simulink model "RobustFormationControl_FractionalModel_under_Dis"  (R2023a)
settings: Solver=ode3  StartTime=0.0  StopTime=30  FixedStep=0.0001  RelTol=1e-3
InitFcn:
  | % close all;
  | % clear all;
  | % clc;
  | % System & Qaudrotor Parameters
  | %==============================
  | m = 0.486;                                         % Quadrotor Mass ( kg )
  | 
  | L = 0.25;                                         % Length of the arm ( m )
  | % L = 0.25;                                         % Length of the arm ( m )
  | 
  | Ixx = 4.856e-03; Iyy = 4.856e-03; Izz = 8.801e-03; % The moments of inertia around x,y and z axes respectively ( kg.m^2 )
  | % Ixx = 3.8278e-03; Iyy = 3.8278e-03; Izz = 7.6566e-03; % The moments of inertia around x,y and z axes respectively ( kg.m^2 )
  | 
  | Jr = 2.8385e-5;                                            % The inertia moment of rotor ( kg.m^2 )
  | % Jr = 0;
  | 
  | % Kx=5.5670e-4;
  | % Ky=5.5670e-4;
  | % Kz=6.3540e-4;
  | % kx=0.032;
  | % ky=0.032;
  | % kz=0.048;
  | Kfx = 5.5670e-4; Kfy = 5.5670e-4; Kfz = 6.3540e-4;% The Rotational drag cofficients ( N/rad/s )
  | 
  | % Ktx = 0.032; Kty = 0.032; Ktz = 0.048;               % The linear drag coefficients in x, y, z respectively ( N/m/s )
  | Ktx = 5.5670e-4; Kty =5.5670e-4; Ktz = 6.3540e-4;               % The linear drag coefficients in x, y, z respectively ( N/m/s )
  | 
  | b = 2.923e-05;                                      % The lift coefficient
  | % b = 2.9842e-05;                                      % The lift coefficient
  | 
  | d = 1.12e-06;                                       % The drag coefficient
  | % d = 3.2320e-07;                                       % The drag coefficient
  | 
  | g = 9.81;                                          % The acceleration due to gravity ( m/s^2 )
  | 
  | %-------- The Coefficients of Non-linear Equations of Quadrotor ( Page 11) -------
  | %--------------------------------------------------------------------------------
  | % Rotational Equations
  | %=====================
  | % Coefficients in ( eq1 ) >>..
  | a1 = (Iyy - Izz)/Ixx;
  | b1 = - Jr/Ixx;
  | c1 = - Kfx/Ixx;
  | d1 = L/Ixx;
  | 
  | % Coefficients in ( eq2 ) >>..
  | a2 = (Izz - Ixx)/Iyy;
  | b2 = Jr/Iyy;
  | c2 = - Kfy/Iyy;
  | d2 = L/Iyy;
  | 
  | % Coefficients in ( eq3 ) >>..
  | a3 = (Ixx - Iyy)/Izz;
  | b3 = - Kfz/Izz;
  | c3 = 1/Izz;
  | % c3 = d/Izz;
  | 
  | % Translational Equations
  | %========================
  | % Coefficients in ( eq4 ) >>..
  | ... (+151 lines)
libraries: fod x135, eeStairGenerator x5
(part 9 of 10)

== system RobustFormationControl_FractionalModel_under_Dis/Fractional Leader with four followers/Follower 4 System/Follower 2 Quadrotor Model/Control Module1/Subsystem5/Subsystem2 ==
  x5 : Inport
  xd5 : Inport  Port=2
  x6 : Inport  Port=3
  xd6 : Inport  Port=4
  S6 : Inport  Port=5
  Abs : Abs  SaturateOnIntegerOverflow=off
  Divide{,1..4} (5 alike) : Product  Inputs=**  RndMeth=Zero  SaturateOnIntegerOverflow=on
  Gain : Gain  Gain=q0
  Gain1 : Gain  Gain=q1
  Gain2 : Gain  Gain=q2
  Integrator : Integrator
  Integrator1 : Integrator
  Integrator2 : Integrator
  Sum1 : Sum  Inputs=+-
  Sum2 : Sum  Inputs=----
  Sum3 : Sum  Inputs=+-
  Tanh : Trigonometry  Operator=tanh
  w : Constant  Value=w
  D3 : Outport  VectorParamsAs1DForOutWhenUnconnected=off
  wires:
  xd6/1 -> Sum1/2
  xd5/1 -> Sum3/2
  x5/1 -> Sum3/1
  x6/1 -> Sum1/1
  S6/1 -> [S6], Abs/1
  Sum1/1 -> [e2]
  Sum3/1 -> [e1]
  Gain/1 -> Integrator/1
  Integrator/1 -> Sum2/1  "B0"
  [e1] -> Divide/2
  Gain1/1 -> Integrator1/1
  Divide/1 -> Gain1/1
  Divide1/1 -> Gain2/1
  Gain2/1 -> Integrator2/1
  [e2] -> Divide1/2
  Abs/1 -> Divide1/1, Divide/1, Gain/1
  Integrator1/1 -> Divide3/2  "B1"
  w/1 -> Sum2/4
  Tanh/1 -> Divide2/2
  [S6] -> Tanh/1
  Divide2/1 -> D3/1
  [e1] -> Divide3/1
  [e2] -> Divide4/1
  Integrator2/1 -> Divide4/2  "B2"
  Divide3/1 -> Sum2/2
  Divide4/1 -> Sum2/3
  Sum2/1 -> Divide2/1

== system RobustFormationControl_FractionalModel_under_Dis/Fractional Leader with four followers/Follower 4 System/Follower 2 Quadrotor Model/Control Module1/Subsystem6/Subsystem3 ==
  xL : Inport
  x7 : Inport  Port=2
  x8 : Inport  Port=3
  dX : Inport  Port=4
  S8 : Inport  Port=5
  Constant : Constant  Value=p/q
  Constant1 : Constant  Value=gx-1
  Derivative : Derivative
  Derivative1 : Derivative
  Divide : Product  Inputs=**  RndMeth=Zero  SaturateOnIntegerOverflow=on
  Fractional derivative : fod/Fractional derivative  gam=alpha1(1)  ww=[0.001; 1000]  n=5  nFod=off
      settings: SourceProductName=FOMCON Toolbox
  Fractional integrator1 : fod/Fractional integrator  gam=alpha2(1)  ww=[0.001; 1000]  n=5  nFod=off
      settings: SourceProductName=FOMCON Toolbox
  Gain : Gain  Gain=cx1
  Gain1 : Gain  Gain=cx2
  Gain2 : Gain  Gain=gx
  Gain3 : Gain  Gain=Sigma1X
  Gain4 : Gain  Gain=Sigma2X
  Power : Math  Operator=pow
  Power1 : Math  Operator=pow
  Sum : Sum
  Sum1 : Sum  Inputs=+--
  Sum2 : Sum  Inputs=+++
  Sum3 : Sum  Inputs=+--
  Tanh : Trigonometry  Operator=tanh
  D2 : Outport  VectorParamsAs1DForOutWhenUnconnected=off
  wires:
  Sum3/1 -> Power1/1, Power/1
  Constant/1 -> Power/2
  Power/1 -> Gain/1
  Gain/1 -> Fractional derivative/1
  Constant1/1 -> Power1/2
  Power1/1 -> Divide/2
  Divide/1 -> Gain1/1
  Gain1/1 -> Gain2/1
  Sum1/1 -> Divide/1
  Gain2/1 -> Fractional integrator1/1
  S8/1 -> Tanh/1, Gain4/1
  Tanh/1 -> Gain3/1
  Gain3/1 -> Sum/1
  Gain4/1 -> Sum/2
  Sum/1 -> Sum2/3
  Fractional derivative/1 -> Sum2/1
  Fractional integrator1/1 -> Sum2/2
  Sum2/1 -> D2/1
  xL/1 -> Sum3/1, Derivative/1
  Derivative/1 -> Sum1/1
  x8/1 -> Sum1/2
  dX/1 -> Sum3/3, Derivative1/1
  Derivative1/1 -> Sum1/3
  x7/1 -> Sum3/2

== system RobustFormationControl_FractionalModel_under_Dis/Fractional Leader with four followers/Follower 4 System/Follower 2 Quadrotor Model/Control Module1/Subsystem6/Subsystem4 ==
  x8 : Inport
  xL : Inport  Port=2
  dX : Inport  Port=3
  Derivative{,1..3} (4 alike) : Derivative
  Divide2 : Product  Inputs=**  RndMeth=Zero  SaturateOnIntegerOverflow=on
  Gain1 : Gain  Commented=on  Gain=a6
  Sum : Sum  Inputs=-+-
  D1 : Outport
  wires:
  Sum/1 -> D1/1
  x8/1 -> Divide2/2
  Divide2/1 -> Sum/1
  [a4D] -> Divide2/1
  Derivative/1 -> Derivative1/1
  xL/1 -> Derivative/1
  Derivative3/1 -> Sum/3
  Derivative2/1 -> Derivative3/1
  dX/1 -> Derivative2/1
  Derivative1/1 -> Sum/2

== system RobustFormationControl_FractionalModel_under_Dis/Fractional Leader with four followers/Follower 4 System/Follower 2 Quadrotor Model/Control Module1/Subsystem6/Subsystem5 ==
  xL : Inport
  x7 : Inport  Port=2
  x8 : Inport  Port=3
  dX : Inport  Port=4
  S8 : Inport  Port=5
  Abs : Abs  SaturateOnIntegerOverflow=off
  Derivative : Derivative
  Derivative1 : Derivative
  Divide{,1..4} (5 alike) : Product  Inputs=**  RndMeth=Zero  SaturateOnIntegerOverflow=on
  Gain : Gain  Gain=q0
  Gain1 : Gain  Gain=q1
  Gain2 : Gain  Gain=q2
  Integrator : Integrator
  Integrator1 : Integrator
  Integrator2 : Integrator
  Sum2 : Sum  Inputs=++++
  Sum4 : Sum  Inputs=+--
  Sum5 : Sum  Inputs=+--
  Tanh : Trigonometry  Operator=tanh
  w : Constant  Value=w
  D3 : Outport  VectorParamsAs1DForOutWhenUnconnected=off
  wires:
  S8/1 -> [S8], Abs/1
  Gain/1 -> Integrator/1
  Integrator/1 -> Sum2/1  "B0"
  [e1] -> Divide/2
  Gain1/1 -> Integrator1/1
  Divide/1 -> Gain1/1
  Divide1/1 -> Gain2/1
  Gain2/1 -> Integrator2/1
  [e2] -> Divide1/2
  Abs/1 -> Divide1/1, Divide/1, Gain/1
  Integrator1/1 -> Divide3/2  "B1"
  w/1 -> Sum2/4
  Tanh/1 -> Divide2/2
  [S8] -> Tanh/1
  Divide2/1 -> D3/1
  [e1] -> Divide3/1
  [e2] -> Divide4/1
  Integrator2/1 -> Divide4/2  "B2"
  Divide3/1 -> Sum2/2
  Divide4/1 -> Sum2/3
  Sum2/1 -> Divide2/1
  Derivative1/1 -> Sum4/3
  Derivative/1 -> Sum4/1
  Sum4/1 -> [e2]
  Sum5/1 -> [e1]
  xL/1 -> Sum5/1, Derivative/1
  x8/1 -> Sum4/2
  dX/1 -> Sum5/3, Derivative1/1
  x7/1 -> Sum5/2

== system RobustFormationControl_FractionalModel_under_Dis/Fractional Leader with four followers/Follower 4 System/Follower 2 Quadrotor Model/Control Module1/Subsystem8/Subsystem ==
  x3 : Inport
  xd3 : Inport  Port=2
  x4 : Inport  Port=3
  xd4 : Inport  Port=4
  S4 : Inport  Port=5
  Constant : Constant  Value=p/q
  Constant1 : Constant  Value=gammaP(2)-1
  Divide : Product  Inputs=**  RndMeth=Zero  SaturateOnIntegerOverflow=on
  Fractional derivative : fod/Fractional derivative  gam=alpha1(2)  ww=[0.001; 1000]  n=5  nFod=off
      settings: SourceProductName=FOMCON Toolbox
  Fractional integrator1 : fod/Fractional integrator  gam=alpha2(2)  ww=[0.001; 1000]  n=5  nFod=off
      settings: SourceProductName=FOMCON Toolbox
  Gain : Gain  Gain=cTheta1
  Gain1 : Gain  Gain=cTheta2
  Gain2 : Gain  Gain=gammaP(2)
  Gain3 : Gain  Gain=Sigma1Theta
  Gain4 : Gain  Gain=Sigma2Theta
  Power : Math  Operator=pow
  Power1 : Math  Operator=pow
  Sum : Sum
  Sum1 : Sum  Inputs=+-
  Sum2 : Sum  Inputs=---
  Sum3 : Sum  Inputs=+-
  Tanh : Trigonometry  Operator=tanh
  D2 : Outport  VectorParamsAs1DForOutWhenUnconnected=off
  wires:
  xd4/1 -> Sum1/2
  xd3/1 -> Sum3/2
  x3/1 -> Sum3/1
  x4/1 -> Sum1/1
  Sum3/1 -> Power1/1, Power/1
  Constant/1 -> Power/2
  Power/1 -> Gain/1
  Gain/1 -> Fractional derivative/1
  Constant1/1 -> Power1/2
  Power1/1 -> Divide/2
  Divide/1 -> Gain1/1
  Gain1/1 -> Gain2/1
  Sum1/1 -> Divide/1
  Gain2/1 -> Fractional integrator1/1
  S4/1 -> Tanh/1, Gain4/1
  Tanh/1 -> Gain3/1
  Gain3/1 -> Sum/1
  Gain4/1 -> Sum/2
  Sum/1 -> Sum2/3
  Fractional derivative/1 -> Sum2/1
  Fractional integrator1/1 -> Sum2/2
  Sum2/1 -> D2/1

== system RobustFormationControl_FractionalModel_under_Dis/Fractional Leader with four followers/Follower 4 System/Follower 2 Quadrotor Model/Control Module1/Subsystem8/Subsystem1 ==
  x4 : Inport
  x6 : Inport  Port=2
  x2 : Inport  Port=3
  Omega : Inport  Port=4
  xd4 : Inport  Port=5
  Gain1 : Gain  Gain=a2
  Gain2 : Gain  Gain=c2
  Gain3 : Gain  Gain=b2
  Math Function1 : Math  Operator=square  SignedPower=on
  Product2 : Product
  Product4 : Product
  Sum3 : Sum  Inputs=---+
  D1 : Outport
  wires:
  x6/1 -> Product2/2
  Gain1/1 -> Sum3/1  "a1 x4 x6"
  Sum3/1 -> D1/1
  Math Function1/1 -> Gain2/1  "x2^2"
  x2/1 -> Product4/1, Product2/1
  x4/1 -> Math Function1/1
  xd4/1 -> Sum3/4
  Product4/1 -> Gain3/1
  Omega/1 -> Product4/2
  Product2/1 -> Gain1/1
  Gain3/1 -> Sum3/3
  Gain2/1 -> Sum3/2  "c1 x2^2"

== system RobustFormationControl_FractionalModel_under_Dis/Fractional Leader with four followers/Follower 4 System/Follower 2 Quadrotor Model/Control Module1/Subsystem8/Subsystem2 ==
  x3 : Inport
  xd3 : Inport  Port=2
  x4 : Inport  Port=3
  xd4 : Inport  Port=4
  S4 : Inport  Port=5
  Abs : Abs  SaturateOnIntegerOverflow=off
  Divide{,1..4} (5 alike) : Product  Inputs=**  RndMeth=Zero  SaturateOnIntegerOverflow=on
  Gain : Gain  Gain=q0
  Gain1 : Gain  Gain=q1
  Gain2 : Gain  Gain=q2
  Integrator : Integrator
  Integrator1 : Integrator
  Integrator2 : Integrator
  Sum1 : Sum  Inputs=+-
  Sum2 : Sum  Inputs=----
  Sum3 : Sum  Inputs=+-
  Tanh : Trigonometry  Operator=tanh
  w : Constant  Value=w
  D3 : Outport  VectorParamsAs1DForOutWhenUnconnected=off
  wires:
  xd4/1 -> Sum1/2
  xd3/1 -> Sum3/2
  x3/1 -> Sum3/1
  x4/1 -> Sum1/1
  S4/1 -> [S4], Abs/1
  Sum1/1 -> [e2]
  Sum3/1 -> [e1]
  Gain/1 -> Integrator/1
  Integrator/1 -> Sum2/1  "B0"
  [e1] -> Divide/2
  Gain1/1 -> Integrator1/1
  Divide/1 -> Gain1/1
  Divide1/1 -> Gain2/1
  Gain2/1 -> Integrator2/1
  [e2] -> Divide1/2
  Abs/1 -> Divide1/1, Divide/1, Gain/1
  Integrator1/1 -> Divide3/2  "B1"
  w/1 -> Sum2/4
  Tanh/1 -> Divide2/2
  [S4] -> Tanh/1
  Divide2/1 -> D3/1
  [e1] -> Divide3/1
  [e2] -> Divide4/1
  Integrator2/1 -> Divide4/2  "B2"
  Divide3/1 -> Sum2/2
  Divide4/1 -> Sum2/3
  Sum2/1 -> Divide2/1

== system RobustFormationControl_FractionalModel_under_Dis/Fractional Leader with four followers/Follower 4 System/Follower 2 Quadrotor Model/Quadrotor Dynamic System/Rotational System/Equation1 ==
  x4 : Inport
  x6 : Inport  Port=2
  U2 : Inport  Port=3
  Omega : Inport  Port=4
  Gain : Gain  Gain=a1
  Gain1 : Gain  Gain=c1
  Gain2 : Gain  Gain=b1
  Gain3 : Gain  Gain=d1
  Integrator : Integrator
  Integrator1 : Integrator
  Math Function : Math  Operator=square  SignedPower=on
  Product : Product
  Product1 : Product
  Sum : Sum  Inputs=|++++
  x1 = Phi : Outport  VectorParamsAs1DForOutWhenUnconnected=off
  x2 : Outport  Port=2  VectorParamsAs1DForOutWhenUnconnected=off
  wires:
  Math Function/1 -> Gain1/1  "x2^2"
  x4/1 -> Product1/1, Product/1
  Integrator/1 -> Math Function/1, x2/1, Integrator1/1
  U2/1 -> Gain3/1
  Gain2/1 -> Sum/3
  Gain3/1 -> Sum/4
  Gain/1 -> Sum/1  "a1 x4 x6"
  Product1/1 -> Gain2/1
  Gain1/1 -> Sum/2  "c1 x2^2"
  Integrator1/1 -> x1 = Phi/1
  Product/1 -> Gain/1
  x6/1 -> Product/2
  Sum/1 -> Integrator/1
  Omega/1 -> Product1/2

== system RobustFormationControl_FractionalModel_under_Dis/Fractional Leader with four followers/Follower 4 System/Follower 2 Quadrotor Model/Quadrotor Dynamic System/Rotational System/Equation2 ==
  x2 : Inport
  x6 : Inport  Port=2
  U3 : Inport  Port=3
  Omega : Inport  Port=4
  Gain : Gain  Gain=a2
  Gain1 : Gain  Gain=c2
  Gain2 : Gain  Gain=b2
  Gain3 : Gain  Gain=d2
  Integrator : Integrator
  Integrator1 : Integrator
  Math Function : Math  Operator=square  SignedPower=on
  Product : Product
  Product1 : Product
  Sum : Sum  Inputs=|++++
  x3 =Theta : Outport  VectorParamsAs1DForOutWhenUnconnected=off
  x4 : Outport  Port=2  VectorParamsAs1DForOutWhenUnconnected=off
  wires:
  Math Function/1 -> Gain1/1  "x4^2"
  x2/1 -> Product1/1, Product/1
  Integrator/1 -> Math Function/1, x4/1, Integrator1/1
  U3/1 -> Gain3/1
  Gain2/1 -> Sum/3
  Gain3/1 -> Sum/4
  Gain/1 -> Sum/1  "a2 x2 x6"
  Product1/1 -> Gain2/1
  Gain1/1 -> Sum/2  "c2 x2^2"
  Integrator1/1 -> x3 =Theta/1
  Product/1 -> Gain/1
  x6/1 -> Product/2
  Sum/1 -> Integrator/1
  Omega/1 -> Product1/2

== system RobustFormationControl_FractionalModel_under_Dis/Fractional Leader with four followers/Follower 4 System/Follower 2 Quadrotor Model/Quadrotor Dynamic System/Rotational System/Equation3 ==
  x2 : Inport
  x4 : Inport  Port=2
  U4 : Inport  Port=3
  Gain : Gain  Gain=a3
  Gain1 : Gain  Gain=b3
  Gain3 : Gain  Gain=c3
  Integrator : Integrator
  Integrator1 : Integrator
  Math Function : Math  Operator=square  SignedPower=on
  Product : Product
  Sum : Sum  Inputs=|+++
  x5 =Psi : Outport  VectorParamsAs1DForOutWhenUnconnected=off
  x6 : Outport  Port=2  VectorParamsAs1DForOutWhenUnconnected=off
  wires:
  Math Function/1 -> Gain1/1  "x6^2"
  x2/1 -> Product/1
  Integrator/1 -> Math Function/1, x6/1, Integrator1/1
  U4/1 -> Gain3/1
  Gain3/1 -> Sum/3
  Gain/1 -> Sum/1  "a3 x2 x4"
  Gain1/1 -> Sum/2  "b3 x6^2"
  Integrator1/1 -> x5 =Psi/1
  Product/1 -> Gain/1
  x4/1 -> Product/2
  Sum/1 -> Integrator/1

== system RobustFormationControl_FractionalModel_under_Dis/Fractional Leader with four followers/Follower 4 System/Follower 2 Quadrotor Model/Quadrotor Dynamic System/Translational System/Equation4 ==
  U1 : Inport
  Ux : Inport  Port=2
  Gain : Gain  Gain=1/m
  Gain1 : Gain  Gain=a4
  Integrator : Integrator
  Integrator1 : Integrator  InitialCondition=4
  Product : Product
  Sum : Sum  Inputs=|++
  x7 = x : Outport  VectorParamsAs1DForOutWhenUnconnected=off
  x8 = xdot : Outport  Port=2  VectorParamsAs1DForOutWhenUnconnected=off
  wires:
  Integrator/1 -> Gain1/1, x8 = xdot/1, Integrator1/1
  U1/1 -> Product/1
  Gain/1 -> Sum/1  "U1 Ux / m"
  Gain1/1 -> Sum/2  "a4 x8"
  Integrator1/1 -> x7 = x/1
  Product/1 -> Gain/1
  Ux/1 -> Product/2
  Sum/1 -> Integrator/1

== system RobustFormationControl_FractionalModel_under_Dis/Fractional Leader with four followers/Follower 4 System/Follower 2 Quadrotor Model/Quadrotor Dynamic System/Translational System/Equation5 ==
  U1 : Inport
  Uy : Inport  Port=2
  Gain : Gain  Gain=1/m
  Gain1 : Gain  Gain=a5
  Integrator : Integrator
  Integrator1 : Integrator  InitialCondition=4
  Product : Product
  Sum : Sum  Inputs=|++
  x9 = y : Outport  VectorParamsAs1DForOutWhenUnconnected=off
  x10 = ydot : Outport  Port=2  VectorParamsAs1DForOutWhenUnconnected=off
  wires:
  Integrator/1 -> x10 = ydot/1, Integrator1/1, Gain1/1
  U1/1 -> Product/1
  Gain/1 -> Sum/1  "U1 Ux / m"
  Gain1/1 -> Sum/2  "a4 x10"
  Integrator1/1 -> x9 = y/1
  Product/1 -> Gain/1
  Uy/1 -> Product/2
  Sum/1 -> Integrator/1

== system RobustFormationControl_FractionalModel_under_Dis/Fractional Leader with four followers/Follower 4 System/Follower 2 Quadrotor Model/Quadrotor Dynamic System/Translational System/Equation6 ==
  U1 : Inport
  x1 : Inport  Port=2
  x3 : Inport  Port=3
  Constant : Constant  Value=g
  Gain : Gain  Gain=1/m
  Gain1 : Gain  Gain=a6
  Integrator : Integrator
  Integrator1 : Integrator
  Product : Product
  Product1 : Product
  Sum : Sum  Inputs=|++-
  Trigonometric Function : Trigonometry  Operator=cos
  Trigonometric Function1 : Trigonometry  Operator=cos
  x11 = z : Outport  VectorParamsAs1DForOutWhenUnconnected=off
  x12 = zdot : Outport  Port=2  VectorParamsAs1DForOutWhenUnconnected=off
  wires:
  U1/1 -> Product/1
  Gain/1 -> Sum/1  "U1 cx1 cx3  / m"
  Gain1/1 -> Sum/2  "a6 x12"
  Integrator1/1 -> x11 = z/1
  Product/1 -> Gain/1
  Sum/1 -> Integrator/1
  Product1/1 -> Product/2
  Trigonometric Function/1 -> Product1/1
  Trigonometric Function1/1 -> Product1/2
  x1/1 -> Trigonometric Function/1
  x3/1 -> Trigonometric Function1/1
  Constant/1 -> Sum/3
  Integrator/1 -> Gain1/1, x12 = zdot/1, Integrator1/1

== system RobustFormationControl_FractionalModel_under_Dis/Fractional Leader with four followers/Fractional Model of the Leader/Fractional Model/Control Module1/Desired System/Desired Values ==
  ft : Inport
  Circular Trajectry : Subsystem  Commented=on
  Helical Trajectry1 : Subsystem
  Step : Step  Time=0  After=0.001  SampleTime=0
  Step Inputs Trajectry : Subsystem  Commented=on
  Phi_d : Outport  VectorParamsAs1DForOutWhenUnconnected=off
  Theta_d : Outport  Port=2  VectorParamsAs1DForOutWhenUnconnected=off
  Psi_d : Outport  Port=3  VectorParamsAs1DForOutWhenUnconnected=off
  Xd : Outport  Port=4  VectorParamsAs1DForOutWhenUnconnected=off
  Yd : Outport  Port=5  VectorParamsAs1DForOutWhenUnconnected=off
  Zd : Outport  Port=6  VectorParamsAs1DForOutWhenUnconnected=off
  wires:
  ft/1 -> Helical Trajectry1/1(t), Circular Trajectry/1(t)
  Step/1 -> Theta_d/1, Phi_d/1
  Helical Trajectry1/1(xd) -> Xd/1
  Helical Trajectry1/3(zd) -> Zd/1
  Helical Trajectry1/2(yd) -> Yd/1
  Helical Trajectry1/4(Psi_d) -> Psi_d/1

== system RobustFormationControl_FractionalModel_under_Dis/Fractional Leader with four followers/Fractional Model of the Leader/Fractional Model/Control Module1/Omega Equations/Control Inputs ==
  w1_sqt : Inport
  w2_sqt : Inport  Port=2
  w3_sqt : Inport  Port=3
  w4_sqt : Inport  Port=4
  Add4 : Sum  Inputs=+-+-
  Omega : Outport  VectorParamsAs1DForOutWhenUnconnected=off
  wires:
  Add4/1 -> Omega/1
  w1_sqt/1 -> Add4/1
  w2_sqt/1 -> Add4/2
  w3_sqt/1 -> Add4/3
  w4_sqt/1 -> Add4/4

== system RobustFormationControl_FractionalModel_under_Dis/Fractional Leader with four followers/Fractional Model of the Leader/Fractional Model/Control Module1/Subsystem/Subsystem ==
  Ux : Inport
  Uy : Inport  Port=2
  Psi_d : Inport  Port=3
  Product : Product
  Product1 : Product
  Subtract : Sum  Inputs=+-
  Trigonometric Function : Trigonometry
  Trigonometric Function1 : Trigonometry  Operator=cos
  Trigonometric Function2 : Trigonometry  Operator=asin
  Phi_d : Outport  VectorParamsAs1DForOutWhenUnconnected=off
  wires:
  Product1/1 -> Subtract/2
  Uy/1 -> Product1/2
  Ux/1 -> Product/1
  Trigonometric Function1/1 -> Product1/1
  Psi_d/1 -> Trigonometric Function1/1, Trigonometric Function/1
  Product/1 -> Subtract/1
  Subtract/1 -> Trigonometric Function2/1
  Trigonometric Function/1 -> Product/2
  Trigonometric Function2/1 -> Phi_d/1

== system RobustFormationControl_FractionalModel_under_Dis/Fractional Leader with four followers/Fractional Model of the Leader/Fractional Model/Control Module1/Subsystem/Subsystem1 ==
  Ux : Inport
  Uy : Inport  Port=2
  Psi_d : Inport  Port=3
  Phi_d : Inport  Port=4
  Constant : Constant
  Divide : Product  Inputs=*/
  Product : Product
  Product1 : Product
  Product2 : Product
  Subtract : Sum
  Trigonometric Function : Trigonometry  Operator=cos
  Trigonometric Function1 : Trigonometry
  Trigonometric Function2 : Trigonometry  Operator=asin
  Trigonometric Function3 : Trigonometry  Operator=cos
  Theta_d : Outport  VectorParamsAs1DForOutWhenUnconnected=off
  wires:
  Product1/1 -> Subtract/2
  Uy/1 -> Product1/2
  Ux/1 -> Product/1
  Trigonometric Function1/1 -> Product1/1
  Psi_d/1 -> Trigonometric Function1/1, Trigonometric Function/1
  Product/1 -> Subtract/1
  Trigonometric Function/1 -> Product/2
  Trigonometric Function2/1 -> Theta_d/1
  Constant/1 -> Divide/1
  Product2/1 -> Trigonometric Function2/1
  Subtract/1 -> Product2/1
  Divide/1 -> Product2/2
  Trigonometric Function3/1 -> Divide/2
  Phi_d/1 -> Trigonometric Function3/1

== system RobustFormationControl_FractionalModel_under_Dis/Fractional Leader with four followers/Fractional Model of the Leader/Fractional Model/Control Module1/Subsystem1/Subsystem ==
  x1 : Inport
  xd1 : Inport  Port=2
  x2 : Inport  Port=3
  xd2 : Inport  Port=4
  Constant : Constant  Value=p/q
  Constant1 : Constant  Value=gammaP(1)
  Divide : Product  Inputs=**  RndMeth=Zero  SaturateOnIntegerOverflow=on
  Fractional integrator : fod/Fractional integrator  gam=alpha1(1)  ww=[0.001; 1000]  n=5  nFod=off
      settings: SourceProductName=FOMCON Toolbox
  Fractional integrator1 : fod/Fractional integrator  gam=alpha2(1)  ww=[0.001; 1000]  n=5  nFod=off
      settings: SourceProductName=FOMCON Toolbox
  Gain : Gain  Gain=cPhi1
  Gain1 : Gain  Gain=cPhi2
  Power : Math  Operator=pow
  Power1 : Math  Operator=pow
  Sum1 : Sum  Inputs=+-
  Sum2 : Sum  Inputs=+++
  Sum3 : Sum  Inputs=+-
  Tanh : Trigonometry  Operator=tanh
  S2 : Outport  VectorParamsAs1DForOutWhenUnconnected=off
  wires:
  xd2/1 -> Sum1/2
  Sum2/1 -> S2/1
  xd1/1 -> Sum3/2
  x1/1 -> Sum3/1
  x2/1 -> Sum1/1
  Sum3/1 -> Tanh/1, Power1/1, Power/1
  Constant/1 -> Power/2
  Power/1 -> Gain/1
  Gain/1 -> Fractional integrator/1
  Constant1/1 -> Power1/2
  Tanh/1 -> Divide/1
  Power1/1 -> Divide/2
  Divide/1 -> Gain1/1
  Gain1/1 -> Fractional integrator1/1
  Sum1/1 -> Sum2/1
  Fractional integrator/1 -> Sum2/2
  Fractional integrator1/1 -> Sum2/3

== system RobustFormationControl_FractionalModel_under_Dis/Fractional Leader with four followers/Fractional Model of the Leader/Fractional Model/Control Module1/Subsystem1/Subsystem1 ==
  x3 : Inport
  xd3 : Inport  Port=2
  x4 : Inport  Port=3
  xd4 : Inport  Port=4
  Gain : Gain  Gain=k3
  Gain1 : Gain  Gain=k4
  Sum1 : Sum  Inputs=+-
  Sum2 : Sum
  Sum3 : Sum  Inputs=+-
  S4 : Outport  VectorParamsAs1DForOutWhenUnconnected=off
  wires:
  xd4/1 -> Sum1/2
  Gain1/1 -> Sum2/2
  Sum2/1 -> S4/1
  xd3/1 -> Sum3/2
  Gain/1 -> Sum2/1
  x3/1 -> Sum3/1
  Sum3/1 -> Gain/1
  x4/1 -> Sum1/1
  Sum1/1 -> Gain1/1

== system RobustFormationControl_FractionalModel_under_Dis/Fractional Leader with four followers/Fractional Model of the Leader/Fractional Model/Control Module1/Subsystem1/Subsystem2 ==
  x5 : Inport
  xd5 : Inport  Port=2
  x6 : Inport  Port=3
  xd6 : Inport  Port=4
  Gain : Gain  Gain=k5
  Gain1 : Gain  Gain=k6
  Sum1 : Sum  Inputs=+-
  Sum2 : Sum
  Sum3 : Sum  Inputs=+-
  S6 : Outport  VectorParamsAs1DForOutWhenUnconnected=off
  wires:
  xd6/1 -> Sum1/2
  Gain1/1 -> Sum2/2
  Sum2/1 -> S6/1
  xd5/1 -> Sum3/2
  Gain/1 -> Sum2/1
  x5/1 -> Sum3/1
  Sum3/1 -> Gain/1
  x6/1 -> Sum1/1
  Sum1/1 -> Gain1/1

== system RobustFormationControl_FractionalModel_under_Dis/Fractional Leader with four followers/Fractional Model of the Leader/Fractional Model/Control Module1/Subsystem1/Subsystem3 ==
  x1 : Inport
  xd1 : Inport  Port=2
  x2 : Inport  Port=3
  xd2 : Inport  Port=4
  Gain : Gain  Gain=k1
  Gain1 : Gain  Gain=k2
  Sum1 : Sum  Inputs=+-
  Sum2 : Sum
  Sum3 : Sum  Inputs=+-
  S2 : Outport  VectorParamsAs1DForOutWhenUnconnected=off
  wires:
  Sum1/1 -> Gain1/1
  x2/1 -> Sum1/1
  Sum3/1 -> Gain/1
  x1/1 -> Sum3/1
  Gain/1 -> Sum2/1
  xd1/1 -> Sum3/2
  Sum2/1 -> S2/1
  Gain1/1 -> Sum2/2
  xd2/1 -> Sum1/2

== system RobustFormationControl_FractionalModel_under_Dis/Fractional Leader with four followers/Fractional Model of the Leader/Fractional Model/Control Module1/Subsystem1/Subsystem5 ==
  x3 : Inport
  xd3 : Inport  Port=2
  x4 : Inport  Port=3
  xd4 : Inport  Port=4
  Constant : Constant  Value=p/q
  Constant1 : Constant  Value=gammaP(2)
  Divide : Product  Inputs=**  RndMeth=Zero  SaturateOnIntegerOverflow=on
  Fractional integrator : fod/Fractional integrator  gam=alpha1(2)  ww=[0.001; 1000]  n=5  nFod=off
      settings: SourceProductName=FOMCON Toolbox
  Fractional integrator1 : fod/Fractional integrator  gam=alpha2(2)  ww=[0.001; 1000]  n=5  nFod=off
      settings: SourceProductName=FOMCON Toolbox
  Gain : Gain  Gain=cTheta1
  Gain1 : Gain  Gain=cTheta2
  Power : Math  Operator=pow
  Power1 : Math  Operator=pow
  Sum1 : Sum  Inputs=+-
  Sum2 : Sum  Inputs=+++
  Sum3 : Sum  Inputs=+-
  Tanh : Trigonometry  Operator=tanh
  S4 : Outport  VectorParamsAs1DForOutWhenUnconnected=off
  wires:
  xd4/1 -> Sum1/2
  Sum2/1 -> S4/1
  xd3/1 -> Sum3/2
  x3/1 -> Sum3/1
  x4/1 -> Sum1/1
  Sum3/1 -> Tanh/1, Power1/1, Power/1
  Constant/1 -> Power/2
  Power/1 -> Gain/1
  Gain/1 -> Fractional integrator/1
  Constant1/1 -> Power1/2
  Tanh/1 -> Divide/1
  Power1/1 -> Divide/2
  Divide/1 -> Gain1/1
  Gain1/1 -> Fractional integrator1/1
  Sum1/1 -> Sum2/1
  Fractional integrator/1 -> Sum2/2
  Fractional integrator1/1 -> Sum2/3

== system RobustFormationControl_FractionalModel_under_Dis/Fractional Leader with four followers/Fractional Model of the Leader/Fractional Model/Control Module1/Subsystem1/Subsystem7 ==
  x5 : Inport
  xd5 : Inport  Port=2
  x6 : Inport  Port=3
  xd6 : Inport  Port=4
  Constant : Constant  Value=p/q
  Constant1 : Constant  Value=gammaP(3)
  Divide : Product  Inputs=**  RndMeth=Zero  SaturateOnIntegerOverflow=on
  Fractional integrator : fod/Fractional integrator  gam=alpha1(3)  ww=[0.001; 1000]  n=5  nFod=off
      settings: SourceProductName=FOMCON Toolbox
  Fractional integrator1 : fod/Fractional integrator  gam=alpha2(3)  ww=[0.001; 1000]  n=5  nFod=off
      settings: SourceProductName=FOMCON Toolbox
  Gain : Gain  Gain=cPsi1
  Gain1 : Gain  Gain=cPsi2
  Power : Math  Operator=pow
  Power1 : Math  Operator=pow
  Sum1 : Sum  Inputs=+-
  Sum2 : Sum  Inputs=+++
  Sum3 : Sum  Inputs=+-
  Tanh : Trigonometry  Operator=tanh
  S6 : Outport  VectorParamsAs1DForOutWhenUnconnected=off
  wires:
  xd6/1 -> Sum1/2
  Sum2/1 -> S6/1
  xd5/1 -> Sum3/2
  x5/1 -> Sum3/1
  x6/1 -> Sum1/1
  Sum3/1 -> Tanh/1, Power1/1, Power/1
  Constant/1 -> Power/2
  Power/1 -> Gain/1
  Gain/1 -> Fractional integrator/1
  Constant1/1 -> Power1/2
  Tanh/1 -> Divide/1
  Power1/1 -> Divide/2
  Divide/1 -> Gain1/1
  Gain1/1 -> Fractional integrator1/1
  Sum1/1 -> Sum2/1
  Fractional integrator/1 -> Sum2/2
  Fractional integrator1/1 -> Sum2/3

== system RobustFormationControl_FractionalModel_under_Dis/Fractional Leader with four followers/Fractional Model of the Leader/Fractional Model/Control Module1/Subsystem2/Subsystem2 ==
  x15f : Inport
  x16f : Inport  Port=2
  x17f : Inport  Port=3
  x18f : Inport  Port=4
  x15fd : Inport  Port=5
  x16fd : Inport  Port=6
  x17fd : Inport  Port=7
  x18fd : Inport  Port=8
  S12 : Inport  Port=9
  Abs : Abs  SaturateOnIntegerOverflow=off
  Divide{,1..4} (5 alike) : Product  Inputs=**  RndMeth=Zero  SaturateOnIntegerOverflow=on
  Gain : Gain  Gain=q0
  Gain1 : Gain  Gain=q1
  Gain2 : Gain  Gain=q2
  Integrator : Integrator
  Integrator1 : Integrator
  Integrator2 : Integrator
  Mux : Mux  Inputs=3
  Scope : Scope  NumInputPorts=3
  Sum : Sum  Inputs=+++
  Sum{1,3..5} (4 alike) : Sum  Inputs=+-
  Sum2 : Sum  Inputs=++++
  Tanh : Trigonometry  Operator=tanh
  To Workspace : ToWorkspace  VariableName=fBz  SampleTime=-1
  w : Constant  Value=w
  D : Outport  VectorParamsAs1DForOutWhenUnconnected=off
  wires:
  x15fd/1 -> Sum3/2
  x15f/1 -> Sum3/1
  S12/1 -> [S12], Abs/1
  Sum3/1 -> [e1]
  Gain/1 -> Integrator/1
  Gain1/1 -> Integrator1/1
  Divide/1 -> Gain1/1
  Divide1/1 -> Gain2/1
  Gain2/1 -> Integrator2/1
  [e4] -> Divide1/2
  Abs/1 -> Divide1/1, Divide/1, Gain/1
  Integrator1/1 -> Divide3/2, Scope/2  "B1"
  w/1 -> Sum2/4
  Tanh/1 -> Divide2/2
  [S12] -> Tanh/1
  Divide2/1 -> D/1
  [e4] -> Divide4/1
  Integrator2/1 -> Divide4/2, Scope/3  "B2"
  Sum2/1 -> Divide2/1
  Sum1/1 -> [e2]
  x16f/1 -> Sum1/1
  x16fd/1 -> Sum1/2
  x17fd/1 -> Sum4/2
  x17f/1 -> Sum4/1
  Sum4/1 -> [e3]
  Sum5/1 -> [e4]
  x18f/1 -> Sum5/1
  x18fd/1 -> Sum5/2
  [e1] -> Sum/1
  [e2] -> Sum/2
  [e3] -> Sum/3
  Sum/1 -> Divide3/1, Divide/2
  Mux/1 -> To Workspace/1
  Divide4/1 -> Mux/3, Sum2/3
  Integrator/1 -> Mux/1, Scope/1, Sum2/1  "B0"
  Divide3/1 -> Mux/2, Sum2/2

== system RobustFormationControl_FractionalModel_under_Dis/Fractional Leader with four followers/Fractional Model of the Leader/Fractional Model/Control Module1/Subsystem3/Subsystem2 ==
  x7f : Inport
  x8f : Inport  Port=2
  x9f : Inport  Port=3
  x10f : Inport  Port=4
  x7fd : Inport  Port=5
  x8fd : Inport  Port=6
  x9fd : Inport  Port=7
  x10fd : Inport  Port=8
  S2 : Inport  Port=9
  Abs : Abs  SaturateOnIntegerOverflow=off
  Divide{,1..4} (5 alike) : Product  Inputs=**  RndMeth=Zero  SaturateOnIntegerOverflow=on
  Gain : Gain  Gain=q0
  Gain1 : Gain  Gain=q1
  Gain2 : Gain  Gain=q2
  Integrator : Integrator
  Integrator1 : Integrator
  Integrator2 : Integrator
  Mux : Mux  Inputs=3
  Scope : Scope  NumInputPorts=3
  Sum : Sum  Inputs=+++
  Sum{1,3..5} (4 alike) : Sum  Inputs=+-
  Sum2 : Sum  Inputs=++++
  Tanh : Trigonometry  Operator=tanh
  To Workspace : ToWorkspace  VariableName=fBx  SampleTime=-1
  w : Constant  Value=w
  D : Outport  VectorParamsAs1DForOutWhenUnconnected=off
  wires:
  x7fd/1 -> Sum3/2
  x7f/1 -> Sum3/1
  S2/1 -> [S2], Abs/1
  Sum3/1 -> [e1]
  Gain/1 -> Integrator/1
  Gain1/1 -> Integrator1/1
  Divide/1 -> Gain1/1
  Divide1/1 -> Gain2/1
  Gain2/1 -> Integrator2/1
  [e4] -> Divide1/2
  Abs/1 -> Divide1/1, Divide/1, Gain/1
  Integrator1/1 -> Divide3/2, Scope/2  "B1"
  w/1 -> Sum2/4
  Tanh/1 -> Divide2/2
  [S2] -> Tanh/1
  Divide2/1 -> D/1
  [e4] -> Divide4/1
  Integrator2/1 -> Divide4/2, Scope/3  "B2"
  Sum2/1 -> Divide2/1
  Sum1/1 -> [e2]
  x8f/1 -> Sum1/1
  x8fd/1 -> Sum1/2
  x9fd/1 -> Sum4/2
  x9f/1 -> Sum4/1
  Sum4/1 -> [e3]
  Sum5/1 -> [e4]
  x10f/1 -> Sum5/1
  x10fd/1 -> Sum5/2
  [e1] -> Sum/1
  [e2] -> Sum/2
  [e3] -> Sum/3
  Sum/1 -> Divide3/1, Divide/2
  Mux/1 -> To Workspace/1
  Divide4/1 -> Mux/3, Sum2/3
  Integrator/1 -> Mux/1, Scope/1, Sum2/1  "B0"
  Divide3/1 -> Mux/2, Sum2/2

== system RobustFormationControl_FractionalModel_under_Dis/Fractional Leader with four followers/Fractional Model of the Leader/Fractional Model/Control Module1/Subsystem4/Subsystem2 ==
  x1 : Inport
  xd1 : Inport  Port=2
  x2 : Inport  Port=3
  xd2 : Inport  Port=4
  S2 : Inport  Port=5
  Abs : Abs  SaturateOnIntegerOverflow=off
  Divide{,1..4} (5 alike) : Product  Inputs=**  RndMeth=Zero  SaturateOnIntegerOverflow=on
  Gain : Gain  Gain=q0
  Gain1 : Gain  Gain=q1
  Gain2 : Gain  Gain=q2
  Integrator : Integrator
  Integrator1 : Integrator
  Integrator2 : Integrator
  Scope : Scope  NumInputPorts=3
  Sum1 : Sum  Inputs=+-
  Sum2 : Sum  Inputs=++++
  Sum3 : Sum  Inputs=+-
  Tanh : Trigonometry  Operator=tanh
  w : Constant  Value=w
  D : Outport  VectorParamsAs1DForOutWhenUnconnected=off
  wires:
  xd2/1 -> Sum1/2
  xd1/1 -> Sum3/2
  x1/1 -> Sum3/1
  x2/1 -> Sum1/1
  S2/1 -> [S2], Abs/1
  Sum1/1 -> [e2]
  Sum3/1 -> [e1]
  Gain/1 -> Integrator/1
  Integrator/1 -> Scope/1, Sum2/1  "B0"
  [e1] -> Divide/2
  Gain1/1 -> Integrator1/1
  Divide/1 -> Gain1/1
  Divide1/1 -> Gain2/1
  Gain2/1 -> Integrator2/1
  [e2] -> Divide1/2
  Abs/1 -> Divide1/1, Divide/1, Gain/1
  Integrator1/1 -> Divide3/2, Scope/2  "B1"
  w/1 -> Sum2/4
  Tanh/1 -> Divide2/2
  [S2] -> Tanh/1
  Divide2/1 -> D/1
  [e1] -> Divide3/1
  [e2] -> Divide4/1
  Integrator2/1 -> Divide4/2, Scope/3  "B2"
  Divide3/1 -> Sum2/2
  Divide4/1 -> Sum2/3
  Sum2/1 -> Divide2/1

== system RobustFormationControl_FractionalModel_under_Dis/Fractional Leader with four followers/Fractional Model of the Leader/Fractional Model/Control Module1/Subsystem5/Subsystem2 ==
  x3 : Inport
  xd3 : Inport  Port=2
  x4 : Inport  Port=3
  xd4 : Inport  Port=4
  S4 : Inport  Port=5
  Abs : Abs  SaturateOnIntegerOverflow=off
  Divide{,1..4} (5 alike) : Product  Inputs=**  RndMeth=Zero  SaturateOnIntegerOverflow=on
  Gain : Gain  Gain=q0
  Gain1 : Gain  Gain=q1
  Gain2 : Gain  Gain=q2
  Integrator : Integrator
  Integrator1 : Integrator
  Integrator2 : Integrator
  Scope : Scope  NumInputPorts=3
  Sum1 : Sum  Inputs=+-
  Sum2 : Sum  Inputs=++++
  Sum3 : Sum  Inputs=+-
  Tanh : Trigonometry  Operator=tanh
  w : Constant  Value=w
  D : Outport  VectorParamsAs1DForOutWhenUnconnected=off
  wires:
  xd4/1 -> Sum1/2
  xd3/1 -> Sum3/2
  x3/1 -> Sum3/1
  x4/1 -> Sum1/1
  S4/1 -> [S4], Abs/1
  Sum1/1 -> [e2]
  Sum3/1 -> [e1]
  Gain/1 -> Integrator/1
  Integrator/1 -> Scope/1, Sum2/1  "B0"
  [e1] -> Divide/2
  Gain1/1 -> Integrator1/1
  Divide/1 -> Gain1/1
  Divide1/1 -> Gain2/1
  Gain2/1 -> Integrator2/1
  [e2] -> Divide1/2
  Abs/1 -> Divide1/1, Divide/1, Gain/1
  Integrator1/1 -> Divide3/2, Scope/2  "B1"
  w/1 -> Sum2/4
  Tanh/1 -> Divide2/2
  [S4] -> Tanh/1
  Divide2/1 -> D/1
  [e1] -> Divide3/1
  [e2] -> Divide4/1
  Integrator2/1 -> Divide4/2, Scope/3  "B2"
  Divide3/1 -> Sum2/2
  Divide4/1 -> Sum2/3
  Sum2/1 -> Divide2/1

== system RobustFormationControl_FractionalModel_under_Dis/Fractional Leader with four followers/Fractional Model of the Leader/Fractional Model/Control Module1/Subsystem6/Subsystem2 ==
  x5 : Inport
  xd5 : Inport  Port=2
  x6 : Inport  Port=3
  xd6 : Inport  Port=4
  S6 : Inport  Port=5
  Abs : Abs  SaturateOnIntegerOverflow=off
  Divide{,1..4} (5 alike) : Product  Inputs=**  RndMeth=Zero  SaturateOnIntegerOverflow=on
  Gain : Gain  Gain=q0
  Gain1 : Gain  Gain=q1
  Gain2 : Gain  Gain=q2
  Integrator : Integrator
  Integrator1 : Integrator
  Integrator2 : Integrator
  Scope : Scope  NumInputPorts=3
  Sum1 : Sum  Inputs=+-
  Sum2 : Sum  Inputs=++++
  Sum3 : Sum  Inputs=+-
  Tanh : Trigonometry  Operator=tanh
  w : Constant  Value=w
  D : Outport  VectorParamsAs1DForOutWhenUnconnected=off
  wires:
  xd6/1 -> Sum1/2
  xd5/1 -> Sum3/2
  x5/1 -> Sum3/1
  x6/1 -> Sum1/1
  S6/1 -> [S6], Abs/1
  Sum1/1 -> [e2]
  Sum3/1 -> [e1]
  Gain/1 -> Integrator/1
  Integrator/1 -> Scope/1, Sum2/1  "B0"
  [e1] -> Divide/2
  Gain1/1 -> Integrator1/1
  Divide/1 -> Gain1/1
  Divide1/1 -> Gain2/1
  Gain2/1 -> Integrator2/1
  [e2] -> Divide1/2
  Abs/1 -> Divide1/1, Divide/1, Gain/1
  Integrator1/1 -> Divide3/2, Scope/2  "B1"
  w/1 -> Sum2/4
  Tanh/1 -> Divide2/2
  [S6] -> Tanh/1
  Divide2/1 -> D/1
  [e1] -> Divide3/1
  [e2] -> Divide4/1
  Integrator2/1 -> Divide4/2, Scope/3  "B2"
  Divide3/1 -> Sum2/2
  Divide4/1 -> Sum2/3
  Sum2/1 -> Divide2/1

== system RobustFormationControl_FractionalModel_under_Dis/Fractional Leader with four followers/Fractional Model of the Leader/Fractional Model/Control Module1/Subsystem7/Subsystem2 ==
  x11f : Inport
  x12f : Inport  Port=2
  x13f : Inport  Port=3
  x14f : Inport  Port=4
  x11fd : Inport  Port=5
  x12fd : Inport  Port=6
  x13fd : Inport  Port=7
  x14fd : Inport  Port=8
  S4 : Inport  Port=9
  Abs : Abs  SaturateOnIntegerOverflow=off
  Divide{,1..4} (5 alike) : Product  Inputs=**  RndMeth=Zero  SaturateOnIntegerOverflow=on
  Gain : Gain  Gain=q0
  Gain1 : Gain  Gain=q1
  Gain2 : Gain  Gain=q2
  Integrator : Integrator
  Integrator1 : Integrator
  Integrator2 : Integrator
  Mux : Mux  Inputs=3
  Scope : Scope  NumInputPorts=3
  Sum : Sum  Inputs=+++
  Sum{1,3..5} (4 alike) : Sum  Inputs=+-
  Sum2 : Sum  Inputs=++++
  Tanh : Trigonometry  Operator=tanh
  To Workspace : ToWorkspace  VariableName=fBy  SampleTime=-1
  w : Constant  Value=w
  D : Outport  VectorParamsAs1DForOutWhenUnconnected=off
  wires:
  x11fd/1 -> Sum3/2
  x11f/1 -> Sum3/1
  S4/1 -> [S4], Abs/1
  Sum3/1 -> [e1]
  Gain/1 -> Integrator/1
  Gain1/1 -> Integrator1/1
  Divide/1 -> Gain1/1
  Divide1/1 -> Gain2/1
  Gain2/1 -> Integrator2/1
  [e4] -> Divide1/2
  Abs/1 -> Divide1/1, Divide/1, Gain/1
  Integrator1/1 -> Divide3/2, Scope/2  "B1"
  w/1 -> Sum2/4
  Tanh/1 -> Divide2/2
  [S4] -> Tanh/1
  Divide2/1 -> D/1
  [e4] -> Divide4/1
  Integrator2/1 -> Divide4/2, Scope/3  "B2"
  Sum2/1 -> Divide2/1
  Sum1/1 -> [e2]
  x12f/1 -> Sum1/1
  x12fd/1 -> Sum1/2
  x13fd/1 -> Sum4/2
  x13f/1 -> Sum4/1
  Sum4/1 -> [e3]
  Sum5/1 -> [e4]
  x14f/1 -> Sum5/1
  x14fd/1 -> Sum5/2
  [e1] -> Sum/1
  [e2] -> Sum/2
  [e3] -> Sum/3
  Sum/1 -> Divide3/1, Divide/2
  Mux/1 -> To Workspace/1
  Divide4/1 -> Mux/3, Sum2/3
  Integrator/1 -> Mux/1, Scope/1, Sum2/1  "B0"
  Divide3/1 -> Mux/2, Sum2/2

== system RobustFormationControl_FractionalModel_under_Dis/Fractional Leader with four followers/Fractional Model of the Leader/Fractional Model/Control Module1/Subsystem8/Subsystem1 ==
  xf11 : Inport
  xfd11 : Inport  Port=2
  xf12 : Inport  Port=3
  xfd12 : Inport  Port=4
  xf13 : Inport  Port=5
  xfd13 : Inport  Port=6
  xf14 : Inport  Port=7
  xfd14 : Inport  Port=8
  Gain : Gain  Gain=q11
  Gain1 : Gain  Gain=q12
  Gain2 : Gain  Gain=q13
  Gain3 : Gain  Gain=q14
  Sum{1,3..5} (4 alike) : Sum  Inputs=+-
  Sum2 : Sum  Inputs=++++
  S10 : Outport  VectorParamsAs1DForOutWhenUnconnected=off
  wires:
  xfd12/1 -> Sum1/2
  Sum2/1 -> S10/1
  xfd11/1 -> Sum3/2
  xf11/1 -> Sum3/1
  Sum3/1 -> Gain/1
  xf12/1 -> Sum1/1
  Sum1/1 -> Gain1/1
  xfd13/1 -> Sum5/2
  Sum5/1 -> Gain2/1
  xf14/1 -> Sum4/1
  xf13/1 -> Sum5/1
  Sum4/1 -> Gain3/1
  xfd14/1 -> Sum4/2
  Gain/1 -> Sum2/1
  Gain1/1 -> Sum2/2
  Gain2/1 -> Sum2/3
  Gain3/1 -> Sum2/4

== system RobustFormationControl_FractionalModel_under_Dis/Fractional Leader with four followers/Fractional Model of the Leader/Fractional Model/Control Module1/Subsystem8/Subsystem2 ==
  xf15 : Inport
  xfd15 : Inport  Port=2
  xf16 : Inport  Port=3
  xfd16 : Inport  Port=4
  xf17 : Inport  Port=5
  xfd17 : Inport  Port=6
  xf18 : Inport  Port=7
  xfd18 : Inport  Port=8
  Gain : Gain  Gain=q15
  Gain1 : Gain  Gain=q16
  Gain2 : Gain  Gain=q17
  Gain3 : Gain  Gain=q18
  Sum{1,3..5} (4 alike) : Sum  Inputs=+-
  Sum2 : Sum  Inputs=++++
  S12 : Outport  VectorParamsAs1DForOutWhenUnconnected=off
  wires:
  xfd16/1 -> Sum1/2
  Sum2/1 -> S12/1
  xfd15/1 -> Sum3/2
  xf15/1 -> Sum3/1
  Sum3/1 -> Gain/1
  xf16/1 -> Sum1/1
  Sum1/1 -> Gain1/1
  xfd17/1 -> Sum5/2
  Sum5/1 -> Gain2/1
  xf18/1 -> Sum4/1
  xf17/1 -> Sum5/1
  Sum4/1 -> Gain3/1
  xfd18/1 -> Sum4/2
  Gain/1 -> Sum2/1
  Gain1/1 -> Sum2/2
  Gain2/1 -> Sum2/3
  Gain3/1 -> Sum2/4

== system RobustFormationControl_FractionalModel_under_Dis/Fractional Leader with four followers/Fractional Model of the Leader/Fractional Model/Control Module1/Subsystem8/Subsystem3 ==
  xf7 : Inport
  xfd7 : Inport  Port=2
  xf8 : Inport  Port=3
  xfd8 : Inport  Port=4
  xf9 : Inport  Port=5
  xfd9 : Inport  Port=6
  xf10 : Inport  Port=7
  xfd10 : Inport  Port=8
  Gain : Gain  Gain=q7
  Gain1 : Gain  Gain=q8
  Gain2 : Gain  Gain=q9
  Gain3 : Gain  Gain=q10
  Sum{1,3..5} (4 alike) : Sum  Inputs=+-
  Sum2 : Sum  Inputs=++++
  S8 : Outport  VectorParamsAs1DForOutWhenUnconnected=off
  wires:
  xfd8/1 -> Sum1/2
  Sum2/1 -> S8/1
  xfd7/1 -> Sum3/2
  xf7/1 -> Sum3/1
  Sum3/1 -> Gain/1
  xf8/1 -> Sum1/1
  Sum1/1 -> Gain1/1
  xfd9/1 -> Sum5/2
  Sum5/1 -> Gain2/1
  xf10/1 -> Sum4/1
  xf9/1 -> Sum5/1
  Sum4/1 -> Gain3/1
  xfd10/1 -> Sum4/2
  Gain/1 -> Sum2/1
  Gain1/1 -> Sum2/2
  Gain2/1 -> Sum2/3
  Gain3/1 -> Sum2/4

== system RobustFormationControl_FractionalModel_under_Dis/Fractional Leader with four followers/Fractional Model of the Leader/Fractional Model/Quadrotor Dynamic System/Fractional Translational System/Equation4 ==
  U1 : Inport
  Ux : Inport  Port=2
  Constant : Constant  Value=0
  Divide : Product  Inputs=**  RndMeth=Zero  SaturateOnIntegerOverflow=on
  Divide1 : Product  Inputs=**  RndMeth=Zero  SaturateOnIntegerOverflow=on
  Fractional integrator{,1..3} (4 alike) : fod/Fractional integrator  gam=0.5  ww=[0.001; 1000]  n=5  nFod=off
      settings: SourceProductName=FOMCON Toolbox
  Gain : Gain  Gain=Dis
  Gain1 : Gain  Commented=on  Gain=1/m
  Gain2 : Gain  Gain=1/m
  Gain3 : Gain  Commented=on  Gain=a4
  Product : Product
  Sum : Sum  Inputs=|++
  Sum1 : Sum  Inputs=|++
  Sum2 : Sum
  xf7 : Outport  VectorParamsAs1DForOutWhenUnconnected=off
  xf8 : Outport  Port=2  VectorParamsAs1DForOutWhenUnconnected=off
  xf9 : Outport  Port=3  VectorParamsAs1DForOutWhenUnconnected=off
  xf10 : Outport  Port=4  VectorParamsAs1DForOutWhenUnconnected=off
  wires:
  Fractional integrator/1 -> Divide/2, xf9/1, Fractional integrator3/1
  U1/1 -> Product/1
  Divide/1 -> Sum/2  "a4 xf9"
  Ux/1 -> Product/2
  Fractional integrator1/1 -> xf10/1, Fractional integrator/1
  Fractional integrator3/1 -> xf8/1, Fractional integrator2/1
  Constant/1 -> Sum1/1
  Fractional integrator2/1 -> Sum1/2
  Sum1/1 -> xf7/1
  [Dpx] -> Gain/1
  Gain2/1 -> Sum2/1
  Sum/1 -> Sum2/2
  Sum2/1 -> Fractional integrator1/1
  [a4D] -> Divide/1
  Product/1 -> Divide1/2
  Divide1/1 -> Sum/1  "U1 Ux / m"
  [b4D] -> Divide1/1
  Gain/1 -> Gain2/1

== system RobustFormationControl_FractionalModel_under_Dis/Fractional Leader with four followers/Fractional Model of the Leader/Fractional Model/Quadrotor Dynamic System/Fractional Translational System/Equation5 ==
  U1 : Inport
  Uy : Inport  Port=2
  Divide : Product  Inputs=**  RndMeth=Zero  SaturateOnIntegerOverflow=on
  Divide1 : Product  Inputs=**  RndMeth=Zero  SaturateOnIntegerOverflow=on
  Fractional integrator{1..2,4..5} (4 alike) : fod/Fractional integrator  gam=0.5  ww=[0.001; 1000]  n=5  nFod=off
      settings: SourceProductName=FOMCON Toolbox
  Gain : Gain  Gain=Dis
  Gain1 : Gain  Gain=1/m
  Gain2 : Gain  Commented=on  Gain=1/m
  Gain3 : Gain  Commented=on  Gain=a5
  Product1 : Product
  Sum : Sum
  Sum1 : Sum  Inputs=|++
  xf11 : Outport  VectorParamsAs1DForOutWhenUnconnected=off
  xf12 : Outport  Port=2  VectorParamsAs1DForOutWhenUnconnected=off
  xf13 : Outport  Port=3  VectorParamsAs1DForOutWhenUnconnected=off
  xf14 : Outport  Port=4  VectorParamsAs1DForOutWhenUnconnected=off
  wires:
  Fractional integrator1/1 -> xf11/1
  Fractional integrator5/1 -> xf14/1, Fractional integrator4/1
  Fractional integrator2/1 -> xf12/1, Fractional integrator1/1
  Fractional integrator4/1 -> xf13/1, Divide/2, Fractional integrator2/1
  Divide/1 -> Sum1/2  "a4 x10"
  Product1/1 -> Divide1/2
  Divide1/1 -> Sum1/1  "U1 Ux / m"
  Uy/1 -> Product1/2
  [a5D] -> Divide/1
  U1/1 -> Product1/1
  [b5D] -> Divide1/1
  Sum/1 -> Fractional integrator5/1
  Sum1/1 -> Sum/2
  Gain/1 -> Gain1/1
  [Dpy] -> Gain/1
  Gain1/1 -> Sum/1

== system RobustFormationControl_FractionalModel_under_Dis/Fractional Leader with four followers/Fractional Model of the Leader/Fractional Model/Quadrotor Dynamic System/Fractional Translational System/Equation6 ==
  U1 : Inport
  x1 : Inport  Port=2
  x3 : Inport  Port=3
  Constant : Constant  Value=g
  Divide1 : Product  Inputs=**  RndMeth=Zero  SaturateOnIntegerOverflow=on
  Divide2 : Product  Inputs=**  RndMeth=Zero  SaturateOnIntegerOverflow=on
  Fractional integrator{1..2,4..5} (4 alike) : fod/Fractional integrator  gam=0.5  ww=[0.001; 1000]  n=5  nFod=off
      settings: SourceProductName=FOMCON Toolbox
  Gain : Gain  Gain=Dis
  Gain1 : Gain  Gain=1/m
  Gain2 : Gain  Commented=on  Gain=a6
  Gain3 : Gain  Commented=on  Gain=1/m
  Product : Product
  Product1 : Product
  Sum : Sum  Inputs=|++-
  Sum1 : Sum
  Trigonometric Function : Trigonometry  Operator=cos
  Trigonometric Function1 : Trigonometry  Operator=cos
  xf15 : Outport  VectorParamsAs1DForOutWhenUnconnected=off
  xf16 : Outport  Port=2  VectorParamsAs1DForOutWhenUnconnected=off
  xf17 : Outport  Port=3  VectorParamsAs1DForOutWhenUnconnected=off
  xf18 : Outport  Port=4  VectorParamsAs1DForOutWhenUnconnected=off
  wires:
  Fractional integrator4/1 -> Divide1/2, xf17/1, Fractional integrator2/1
  U1/1 -> Product/1
  Divide2/1 -> Sum/1  "U1 cx1 cx3  / m"
  Divide1/1 -> Sum/2  "a6 x12"
  Fractional integrator1/1 -> xf15/1
  Product/1 -> Divide2/2
  Product1/1 -> Product/2
  Trigonometric Function/1 -> Product1/1
  Trigonometric Function1/1 -> Product1/2
  x1/1 -> Trigonometric Function/1
  x3/1 -> Trigonometric Function1/1
  Constant/1 -> Sum/3
  Fractional integrator5/1 -> xf18/1, Fractional integrator4/1
  Fractional integrator2/1 -> Fractional integrator1/1, xf16/1
  [b6D] -> Divide2/1
  [a6D] -> Divide1/1
  Gain1/1 -> Sum1/1
  [Dpz] -> Gain/1
  Sum/1 -> Sum1/2
  Gain/1 -> Gain1/1
  Sum1/1 -> Fractional integrator5/1

== system RobustFormationControl_FractionalModel_under_Dis/Fractional Leader with four followers/Fractional Model of the Leader/Fractional Model/Quadrotor Dynamic System/Rotational System/Equation1 ==
  x4 : Inport
  x6 : Inport  Port=2
  U2 : Inport  Port=3
  Omega : Inport  Port=4
  Gain : Gain  Commented=on  Gain=a1
  Gain1 : Gain  Commented=on  Gain=c1
  Gain2 : Gain  Commented=on  Gain=b1
  Gain3 : Gain  Commented=on  Gain=d1
  Gain4 : Gain
  Gain5 : Gain  Gain=Dis
  Integrator : Integrator
  Integrator1 : Integrator
  Math Function : Math  Operator=square  SignedPower=on
  Product{,1..5} (6 alike) : Product
  Sum : Sum  Inputs=|++++
  Sum1 : Sum
  x1 = Phi : Outport  VectorParamsAs1DForOutWhenUnconnected=off
  x2 : Outport  Port=2  VectorParamsAs1DForOutWhenUnconnected=off
  wires:
  Math Function/1 -> Product4/2  "x2^2"
  x4/1 -> Product1/1, Product/1
  Integrator/1 -> Math Function/1, x2/1, Integrator1/1
  U2/1 -> Product5/2
  Product3/1 -> Sum/3
  Product5/1 -> Sum/4
  Product2/1 -> Sum/1  "a1 x4 x6"
  Product1/1 -> Product3/2
  Product4/1 -> Sum/2  "c1 x2^2"
  Integrator1/1 -> x1 = Phi/1
  Product/1 -> Product2/2
  x6/1 -> Product/2
  Omega/1 -> Product1/2
  Sum1/1 -> Integrator/1
  [Dphi1] -> Gain5/1
  Sum/1 -> Sum1/2
  Gain4/1 -> Sum1/1
  Gain5/1 -> Gain4/1
  [a1D] -> Product2/1
  [b1D] -> Product3/1
  [c1D] -> Product4/1
  [d1D] -> Product5/1

== system RobustFormationControl_FractionalModel_under_Dis/Fractional Leader with four followers/Fractional Model of the Leader/Fractional Model/Quadrotor Dynamic System/Rotational System/Equation2 ==
  x2 : Inport
  x6 : Inport  Port=2
  U3 : Inport  Port=3
  Omega : Inport  Port=4
  Gain : Gain  Commented=on  Gain=a2
  Gain1 : Gain  Commented=on  Gain=c2
  Gain2 : Gain  Commented=on  Gain=b2
  Gain3 : Gain  Commented=on  Gain=d2
  Gain4 : Gain
  Gain5 : Gain  Gain=Dis
  Integrator : Integrator
  Integrator1 : Integrator
  Math Function : Math  Operator=square  SignedPower=on
  Product{,1..5} (6 alike) : Product
  Sum : Sum  Inputs=|++++
  Sum1 : Sum
  x3 =Theta : Outport  VectorParamsAs1DForOutWhenUnconnected=off
  x4 : Outport  Port=2  VectorParamsAs1DForOutWhenUnconnected=off
  wires:
  Math Function/1 -> Product4/2  "x4^2"
  x2/1 -> Product1/1, Product/1
  Integrator/1 -> Math Function/1, x4/1, Integrator1/1
  U3/1 -> Product5/2
  Product3/1 -> Sum/3
  Product5/1 -> Sum/4
  Product2/1 -> Sum/1  "a2 x2 x6"
  Product1/1 -> Product3/2
  Product4/1 -> Sum/2  "c2 x2^2"
  Integrator1/1 -> x3 =Theta/1
  Product/1 -> Product2/2
  x6/1 -> Product/2
  Omega/1 -> Product1/2
  Sum1/1 -> Integrator/1
  [Dphi2] -> Gain5/1
  Sum/1 -> Sum1/2
  Gain4/1 -> Sum1/1
  Gain5/1 -> Gain4/1
  [a2D] -> Product2/1
  [b2D] -> Product3/1
  [c2D] -> Product4/1
  [d2D] -> Product5/1

== system RobustFormationControl_FractionalModel_under_Dis/Fractional Leader with four followers/Fractional Model of the Leader/Fractional Model/Quadrotor Dynamic System/Rotational System/Equation3 ==
  x2 : Inport
  x4 : Inport  Port=2
  U4 : Inport  Port=3
  Gain : Gain  Commented=on  Gain=a3
  Gain1 : Gain  Commented=on  Gain=b3
  Gain2 : Gain
  Gain3 : Gain  Commented=on  Gain=c3
  Gain4 : Gain  Gain=Dis
  Integrator : Integrator
  Integrator1 : Integrator
  Math Function : Math  Operator=square  SignedPower=on
  Product{,1..3} (4 alike) : Product
  Sum : Sum  Inputs=|+++
  Sum1 : Sum
  x5 =Psi : Outport  VectorParamsAs1DForOutWhenUnconnected=off
  x6 : Outport  Port=2  VectorParamsAs1DForOutWhenUnconnected=off
  wires:
  Math Function/1 -> Product2/2  "x6^2"
  x2/1 -> Product/1
  Integrator/1 -> Math Function/1, x6/1, Integrator1/1
  U4/1 -> Product3/2
  Product3/1 -> Sum/3
  Product1/1 -> Sum/1  "a3 x2 x4"
  Product2/1 -> Sum/2  "b3 x6^2"
  Integrator1/1 -> x5 =Psi/1
  Product/1 -> Product1/2
  x4/1 -> Product/2
  Sum1/1 -> Integrator/1
  [Dphi3] -> Gain4/1
  Sum/1 -> Sum1/2
  Gain2/1 -> Sum1/1
  Gain4/1 -> Gain2/1
  [a3D] -> Product1/1
  [b3D] -> Product2/1
  [c3D] -> Product3/1

== system RobustFormationControl_FractionalModel_under_Dis/Fractional Leader with four followers/Fractional Model of the Leader/Fractional Model/Control Module1/Desired System/Desired Values/Circular Trajectry ==
  t : Inport
  Gain1 : Gain
  Step : Step  Time=0  SampleTime=0
  Step1 : Step  Time=0  SampleTime=0
  Trigonometric Function : Trigonometry  Operator=cos
  Trigonometric Function1 : Trigonometry
  xd : Outport  VectorParamsAs1DForOutWhenUnconnected=off
  yd : Outport  Port=2  VectorParamsAs1DForOutWhenUnconnected=off
  zd : Outport  Port=3  VectorParamsAs1DForOutWhenUnconnected=off
  Psi_d : Outport  Port=4  VectorParamsAs1DForOutWhenUnconnected=off
  wires:
  t/1 -> Gain1/1
  Gain1/1 -> Trigonometric Function1/1, Trigonometric Function/1
  Trigonometric Function/1 -> xd/1
  Trigonometric Function1/1 -> yd/1
  Step/1 -> zd/1
  Step1/1 -> Psi_d/1
